simulink library "filters_lib"  (R2018b)
settings: Solver=VariableStepAuto  StartTime=0.0  StopTime=10.0  RelTol=1e-3
undefined symbols (not defined in the file or in its folder): DiscIntNeverNeededParam
libraries: quatAttitudeController_lib x1, $bdroot x1
settings Model: Creator=Ybeyer  LastModifiedBy=yannic
settings DebuggingCC: LibraryContextMissingDiagnostic=none
settings SFSimCC: SimUseLocalCustomCode=off
settings RTWCC: RTWUseLocalCustomCode=off
settings CodeAppCC: StateflowObjectComments=on

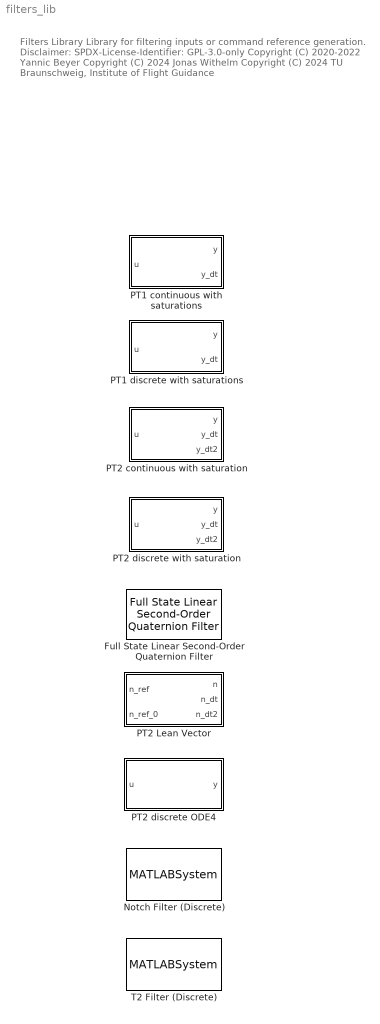
== system filters_lib ==
  note: Filters Library
      |
      | Library for filtering inputs or command reference generation.
      |
      | Disclaimer:
      | SPDX-License-Identifier: GPL-3.0-only
      |
      | Copyright (C) 2020-2022 Yannic Beyer
      | Copyright (C) 2024 Jonas Withelm
      | Copyright (C) 2024 TU Braunschweig, Institute of Flight Guidance
  Full State Linear Second-Order Quaternion Filter : quatAttitudeController_lib/Full State Linear Second-Order Quaternion Filter  omega_0=15  D=1  q_0=[1; 0; 0; 0]  omega_Kb_0=[0; 0; 0]
      settings: SourceProductName=LADAC
  Notch Filter (Discrete) : MATLABSystem  System=NotchFilter  omega_0=2*pi*80  omega_c=2*pi*40  A0_dB=40  Ts=-1  SimulateUsing=Code generation
      mask Type: NotchFilter
      mask Display:
      | disp('NotchFilter');
      | port_label('input',1,'u');
      | port_label('output',1,'y');
  PT1 continuous with saturations : Subsystem  mask{T=1, x_max=inf, x_min=-inf, x_dt_max=inf, x_dt_min=-inf, x_init=0}
      mask prompts: T "Time constant"; x_max "Maximum output"; x_min "Minimum output"; x_dt_max "Maximum output_rate"; x_dt_min "Minimum output rate"; x_init "Initial output"
  PT1 discrete with saturations : Subsystem  mask(PT1 discrete with saturation){param_src=internal, T=1, x_max=inf, x_min=-inf, x_dt_max=inf, x_dt_min=-inf, y_0_src=internal, x_init=0, is_y_dt_checked=on, is_external_reset_checked=off, mask_expr_handling_config=default}
      mask prompts: param_src "Parameter source:"; T "Time constant:"; x_max "Maximum output:"; x_min "Minimum output:"; x_dt_max "Maximum output velocity:"; x_dt_min "Minimum output velocity:"; y_0_src "Initial output source:"; x_init "Initial output:"; is_y_dt_checked "Enable velocity output"; is_external_reset_checked "Enable external reset input"
      mask init:
      | pt1BlockInit(param_src, y_0_src, is_y_dt_checked, is_external_reset_checked);
      | 
      | maskExprHandling(gcbh, mask_expr_handling_config);
      mask TypeOptions param_src: internal | external
      mask TypeOptions y_0_src: internal | external
      mask TypeOptions mask_expr_handling_config: default | passthrough (tunable)
      mask DialogControl TabGeneral Prompt: General
      mask DialogControl TabLimits Prompt: Limits
      mask DialogControl TabInitial Prompt: Initial Values
      mask DialogControl CodeGenerationSettings Prompt: Code Generation Settings
      mask DialogControl maskExprHandlingText Prompt: Mask expression handling
      mask DialogControl maskExprHandlingReadme Prompt: README
      mask DialogControl maskExprHandlingReadme Tooltip: https://github.com/iff-gsc/m-Utils/tree/main/simulink/mask_expression_handling/README.md
      mask DialogControl maskExprHandlingReadme Callback: web('https://github.com/iff-gsc/m-Utils/tree/main/simulink/mask_expression_handling/README.md','-browser')
  PT2 Lean Vector : Subsystem  mask(2nd Order Reduced Attitude Reference Model){param_src=internal, omega=1, d=1, x_max=inf, x_min=-inf, x_dt_max=inf, x_dt_min=-inf, x_dt2_max=inf, x_dt2_min=-inf, n_ref_0_src=external, x_init=[0, 0, -1], n_ref_dt_0_src=internal, x_dt_init=[0, 0, 0], is_n_dt_checked=on, is_n_dt2_checked=on, is_external_reset_checked=off, mask_expr_handling_config=default}
      mask prompts: param_src "Parameter source:"; omega "Natural frequency:"; d "Damping ratio:"; x_max "Maximum output:"; x_min "Minimum output:"; x_dt_max "Maximum output velocity:"; x_dt_min "Minimum output velocity:"; x_dt2_max "Maximum output acceleration:"; x_dt2_min "Minimum output acceleration:"; n_ref_0_src "Initial lean vector source:"; x_init "Initial lean vector:"; n_ref_dt_0_src "Initial velocity source:"; x_dt_init "Initial velocity:"; is_n_dt_checked "Enable velocity output"; is_n_dt2_checked "Enable acceleration output"; is_external_reset_checked "Enable external reset input"
      mask help: The lean vector is filtered by a second order low-pass filter. A unit vector output is assured. Moreover, the derivatives are also adjusted to match with the output unit vector.
      mask init:
      | pt2LeanVectorBlockInit(param_src, n_ref_0_src, n_ref_dt_0_src, is_n_dt_checked, is_n_dt2_checked, is_external_reset_checked);
      | 
      | maskExprHandling(gcbh, mask_expr_handling_config);
      mask TypeOptions param_src: internal | external
      mask TypeOptions n_ref_0_src: internal | external
      mask TypeOptions n_ref_dt_0_src: internal | external
      mask TypeOptions mask_expr_handling_config: default | passthrough (tunable)
      mask DialogControl TabGeneral Prompt: General
      mask DialogControl TabLimits Prompt: Limits
      mask DialogControl TabInitial Prompt: Initial Values
      mask DialogControl CodeGenerationSettings Prompt: Code Generation Settings
      mask DialogControl maskExprHandlingText Prompt: Mask expression handling
      mask DialogControl maskExprHandlingReadme Prompt: README
      mask DialogControl maskExprHandlingReadme Tooltip: https://github.com/iff-gsc/m-Utils/tree/main/simulink/mask_expression_handling/README.md
      mask DialogControl maskExprHandlingReadme Callback: web('https://github.com/iff-gsc/m-Utils/tree/main/simulink/mask_expression_handling/README.md','-browser')
  PT2 continuous with saturation : Subsystem  mask{omega=0.7, d=1, x_dt2_max=inf, x_dt2_min=-inf, x_dt_max=inf, x_dt_min=-inf, x_max=inf, x_min=-inf, x_init=0, x_dt_init=0}
      mask prompts: omega "Natural frequency"; d "Damping ratio"; x_dt2_max "Maximum acceleration"; x_dt2_min "Minimum acceleration"; x_dt_max "Maximum rate"; x_dt_min "Minimum rate"; x_max "Maximum position"; x_min "Minimum position"; x_init "Initial position"; x_dt_init "Initial rate"
  PT2 discrete ODE4 : Subsystem  mask{param_src=internal, omega=1, d=1, y_0_src=internal, x_init=0, y_dt_0_src=internal, x_dt_init=0, is_y_dt_checked=off, is_y_dt2_checked=off, is_external_reset_checked=off, mask_expr_handling_config=default}
      mask prompts: param_src "Parameter source:"; omega "Natural frequency, rad/s:"; d "Damping ratio:"; y_0_src "Initial output source:"; x_init "Initial output:"; y_dt_0_src "Initial velocity source:"; x_dt_init "Initial velocity:"; is_y_dt_checked "Enable velocity output"; is_y_dt2_checked "Enable acceleration output"; is_external_reset_checked "Enable external reset input"
      mask init:
      | pt2BlockInit(param_src, y_0_src, y_dt_0_src, is_y_dt_checked, is_y_dt2_checked, is_external_reset_checked);
      | 
      | maskExprHandling(gcbh, mask_expr_handling_config);
      mask TypeOptions param_src: internal | external
      mask TypeOptions y_0_src: internal | external
      mask TypeOptions y_dt_0_src: internal | external
      mask TypeOptions mask_expr_handling_config: default | passthrough (tunable)
      mask DialogControl DescGroupVar Prompt: Discrete second-order low-pass filter with ODE4 implementation
      mask DialogControl DescTextVar Prompt: This is a discrete second-order low-pass filter implementation with Runge-Kutta (ODE4) integration method. This method is more accurate than the standard Euler forward method (ODE1) and can be useful if the cut-off frequency is high and the sampling frequency is low.
      mask DialogControl TabGeneral Prompt: General
      mask DialogControl TabInitial Prompt: Initial Values
      mask DialogControl CodeGenerationSettings Prompt: CodeGenerationSettings
      mask DialogControl maskExprHandlingText Prompt: Mask expression handling
      mask DialogControl maskExprHandlingReadme Prompt: README
  PT2 discrete with saturation : Subsystem  mask(PT2 discrete with saturation){param_src=internal, omega=1, d=0.7, x_max=inf, x_min=-inf, x_dt_max=inf, x_dt_min=-inf, x_dt2_max=inf, x_dt2_min=-inf, y_0_src=internal, x_init=0, y_dt_0_src=internal, x_dt_init=0, is_y_dt_checked=on, is_y_dt2_checked=on, is_external_reset_checked=off, mask_expr_handling_config=default}
      mask prompts: param_src "Parameter source:"; omega "Natural frequency:"; d "Damping ratio:"; x_max "Maximum output:"; x_min "Minimum output:"; x_dt_max "Maximum output velocity:"; x_dt_min "Minimum output velocity:"; x_dt2_max "Maximum output acceleration:"; x_dt2_min "Minimum output acceleration:"; y_0_src "Initial output source:"; x_init "Initial output:"; y_dt_0_src "Initial velocity source:"; x_dt_init "Initial velocity:"; is_y_dt_checked "Enable velocity output"; is_y_dt2_checked "Enable acceleration output"; is_external_reset_checked "Enable external reset input"
      mask init:
      | pt2BlockInit(param_src, y_0_src, y_dt_0_src, is_y_dt_checked, is_y_dt2_checked, is_external_reset_checked);
      | 
      | maskExprHandling(gcbh, mask_expr_handling_config);
      mask TypeOptions param_src: internal | external
      mask TypeOptions y_0_src: internal | external
      mask TypeOptions y_dt_0_src: internal | external
      mask TypeOptions mask_expr_handling_config: default | passthrough (tunable)
      mask DialogControl TabGeneral Prompt: General
      mask DialogControl TabLimits Prompt: Limits
      mask DialogControl TabInitial Prompt: Initial Values
      mask DialogControl CodeGenerationSettings Prompt: Code Generation Settings
      mask DialogControl maskExprHandlingText Prompt: Mask expression handling
      mask DialogControl maskExprHandlingReadme Prompt: README
      mask DialogControl maskExprHandlingReadme Tooltip: https://github.com/iff-gsc/m-Utils/tree/main/simulink/mask_expression_handling/README.md
      mask DialogControl maskExprHandlingReadme Callback: web('https://github.com/iff-gsc/m-Utils/tree/main/simulink/mask_expression_handling/README.md','-browser')
  T2 Filter (Discrete) : MATLABSystem  System=T2Filter  omega_0=10  d=0.7  Ts=-1  is_vel=false  is_acc=false  SimulateUsing=Code generation
      mask Type: T2Filter
      mask Display:
      | disp('T2Filter');
      | port_label('input',1,'u');
      | port_label('output',1,'y');

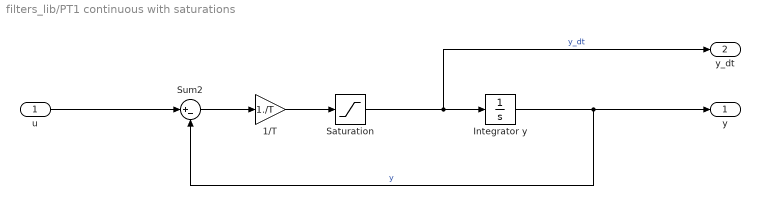
== system filters_lib/PT1 continuous with saturations ==
  u : Inport
  1/T : Gain  Gain=1./T
  Integrator y : Integrator  InitialCondition=x_init  LimitOutput=on  UpperSaturationLimit=x_max  LowerSaturationLimit=x_min
  Saturation : Saturate  UpperLimit=x_dt_max  LowerLimit=x_dt_min
  Sum2 : Sum  Inputs=|+-
  y : Outport
  y_dt : Outport  Port=2
  wires:
  Saturation/1 -> Integrator y/1, y_dt/1  "y_dt"
  Integrator y/1 -> y/1, Sum2/2  "y"
  Sum2/1 -> 1/T/1
  u/1 -> Sum2/1
  1/T/1 -> Saturation/1

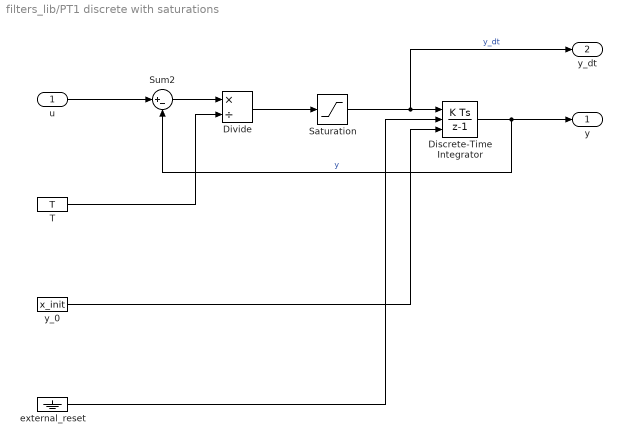
== system filters_lib/PT1 discrete with saturations ==
  u : Inport
  Discrete-Time Integrator : DiscreteIntegrator  ExternalReset=rising  InitialConditionSource=external  InitialCondition=x_init  SampleTime=-1  LimitOutput=on  UpperSaturationLimit=x_max  LowerSaturationLimit=x_min  ICPrevOutput=DiscIntNeverNeededParam  ICPrevScaledInput=DiscIntNeverNeededParam
  Divide : Product  Inputs=*/
  Saturation : Saturate  UpperLimit=x_dt_max  LowerLimit=x_dt_min
  Sum2 : Sum  Inputs=|+-
  T : Constant  Value=T
  external_reset : Ground
  y_0 : Constant  Value=x_init
  y : Outport
  y_dt : Outport  Port=2
  wires:
  Saturation/1 -> y_dt/1, Discrete-Time Integrator/1  "y_dt"
  Discrete-Time Integrator/1 -> y/1, Sum2/2  "y"
  Sum2/1 -> Divide/1
  u/1 -> Sum2/1
  Divide/1 -> Saturation/1
  T/1 -> Divide/2
  y_0/1 -> Discrete-Time Integrator/3
  external_reset/1 -> Discrete-Time Integrator/2

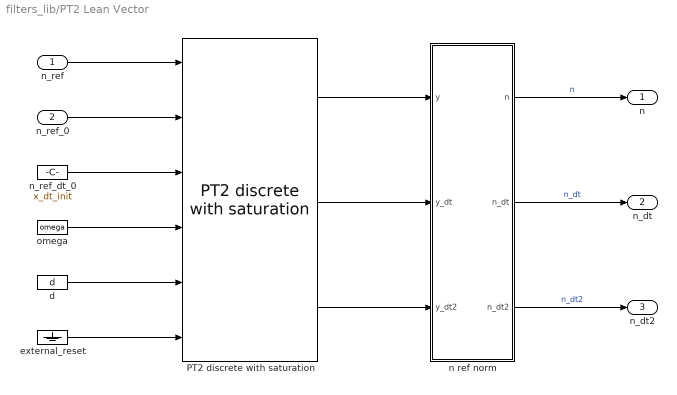
== system filters_lib/PT2 Lean Vector ==
  n_ref : Inport  PortDimensions=3
  n_ref_0 : Inport  Port=2  PortDimensions=3
  PT2 discrete with saturation : $bdroot/PT2 discrete with saturation  param_src=external  omega=omega  d=d  x_max=x_max  x_min=x_min  x_dt_max=x_dt_max  x_dt_min=x_dt_min  x_dt2_max=x_dt2_max  x_dt2_min=x_dt2_min  y_0_src=external  x_init=n_ref_0_src  y_dt_0_src=external  x_dt_init=n_ref_dt_0_src  is_y_dt_checked=on  is_y_dt2_checked=on  is_external_reset_checked=on  mask_expr_handling_config=default
  d : Constant  Value=d
  external_reset : Ground
  n ref norm : MATLAB Function  TreatAsAtomicUnit=on
  n_ref_dt_0 : Constant  Value=x_dt_init
  omega : Constant  Value=omega
  n : Outport  PortDimensions=3
  n_dt : Outport  Port=2  PortDimensions=3
  n_dt2 : Outport  Port=3  PortDimensions=3
  wires:
  n ref norm/3(n_dt2) -> n_dt2/1  "n_dt2"
  n ref norm/2(n_dt) -> n_dt/1  "n_dt"
  n ref norm/1(n) -> n/1  "n"
  PT2 discrete with saturation/1 -> n ref norm/1(y)
  PT2 discrete with saturation/2 -> n ref norm/2(y_dt)
  PT2 discrete with saturation/3 -> n ref norm/3(y_dt2)
  n_ref/1 -> PT2 discrete with saturation/1
  d/1 -> PT2 discrete with saturation/5
  omega/1 -> PT2 discrete with saturation/4
  n_ref_dt_0/1 -> PT2 discrete with saturation/3
  n_ref_0/1 -> PT2 discrete with saturation/2
  external_reset/1 -> PT2 discrete with saturation/6

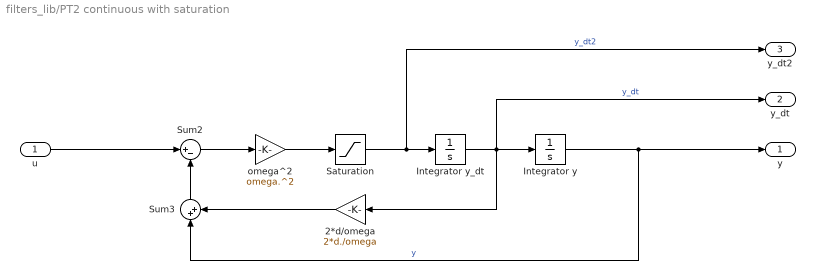
== system filters_lib/PT2 continuous with saturation ==
  u : Inport
  2*d/omega : Gain  Gain=2*d./omega
  Integrator y : Integrator  InitialCondition=x_init  LimitOutput=on  UpperSaturationLimit=x_max  LowerSaturationLimit=x_min
  Integrator y_dt : Integrator  InitialCondition=x_dt_init  LimitOutput=on  UpperSaturationLimit=x_dt_max  LowerSaturationLimit=x_dt_min
  Saturation : Saturate  UpperLimit=x_dt2_max  LowerLimit=x_dt2_min
  Sum2 : Sum  Inputs=|+-
  Sum3 : Sum  Inputs=|++
  omega^2 : Gain  Gain=omega.^2
  y : Outport
  y_dt : Outport  Port=2
  y_dt2 : Outport  Port=3
  wires:
  Integrator y_dt/1 -> y_dt/1, Integrator y/1, 2*d/omega/1  "y_dt"
  Integrator y/1 -> y/1, Sum3/1  "y"
  Sum2/1 -> omega^2/1
  2*d/omega/1 -> Sum3/2
  u/1 -> Sum2/1
  Sum3/1 -> Sum2/2
  omega^2/1 -> Saturation/1
  Saturation/1 -> y_dt2/1, Integrator y_dt/1  "y_dt2"

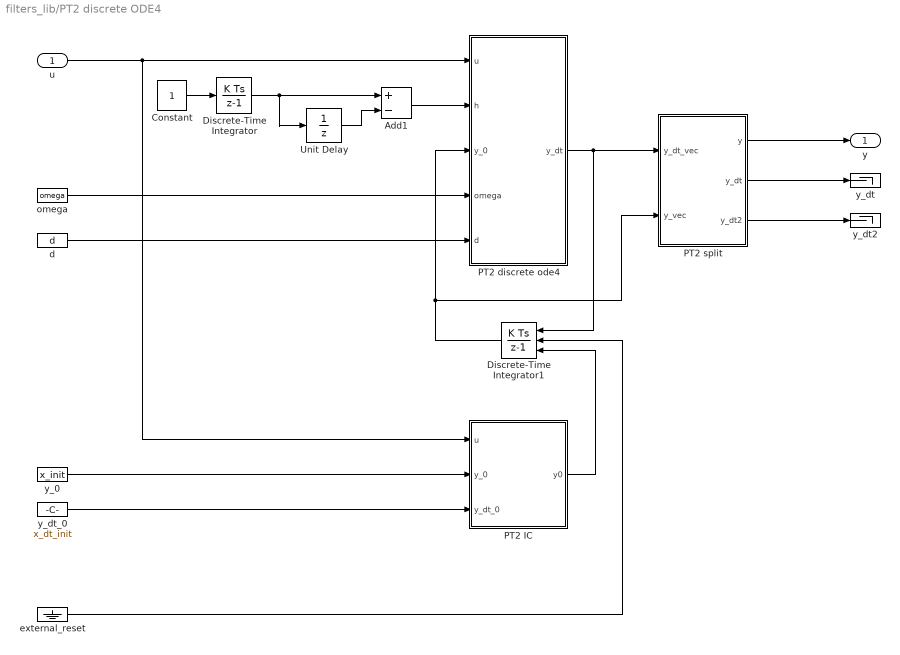
== system filters_lib/PT2 discrete ODE4 ==
  u : Inport
  Add1 : Sum  Inputs=+-
  Constant : Constant
  Discrete-Time Integrator : DiscreteIntegrator  SampleTime=-1  ICPrevOutput=DiscIntNeverNeededParam  ICPrevScaledInput=DiscIntNeverNeededParam
  Discrete-Time Integrator1 : DiscreteIntegrator  ExternalReset=rising  InitialConditionSource=external  SampleTime=-1  ICPrevOutput=DiscIntNeverNeededParam  ICPrevScaledInput=DiscIntNeverNeededParam
  PT2 IC : MATLAB Function  TreatAsAtomicUnit=on
  PT2 discrete ode4 : MATLAB Function  TreatAsAtomicUnit=on
  PT2 split : MATLAB Function  TreatAsAtomicUnit=on
  Unit Delay : UnitDelay  SampleTime=-1
  d : Constant  Value=d
  external_reset : Ground
  omega : Constant  Value=omega
  y_0 : Constant  Value=x_init
  y_dt : Terminator
  y_dt2 : Terminator
  y_dt_0 : Constant  Value=x_dt_init
  y : Outport
  wires:
  u/1 -> PT2 IC/1(u), PT2 discrete ode4/1(u)
  Constant/1 -> Discrete-Time Integrator/1
  Add1/1 -> PT2 discrete ode4/2(h)
  Discrete-Time Integrator/1 -> Add1/1, Unit Delay/1
  Unit Delay/1 -> Add1/2
  omega/1 -> PT2 discrete ode4/4(omega)
  d/1 -> PT2 discrete ode4/5(d)
  PT2 discrete ode4/1(y_dt) -> Discrete-Time Integrator1/1, PT2 split/1(y_dt_vec)
  Discrete-Time Integrator1/1 -> PT2 split/2(y_vec), PT2 discrete ode4/3(y_0)
  PT2 split/1(y) -> y/1
  PT2 split/2(y_dt) -> y_dt/1
  PT2 split/3(y_dt2) -> y_dt2/1
  y_0/1 -> PT2 IC/2(y_0)
  y_dt_0/1 -> PT2 IC/3(y_dt_0)
  external_reset/1 -> Discrete-Time Integrator1/2
  PT2 IC/1(y0) -> Discrete-Time Integrator1/3

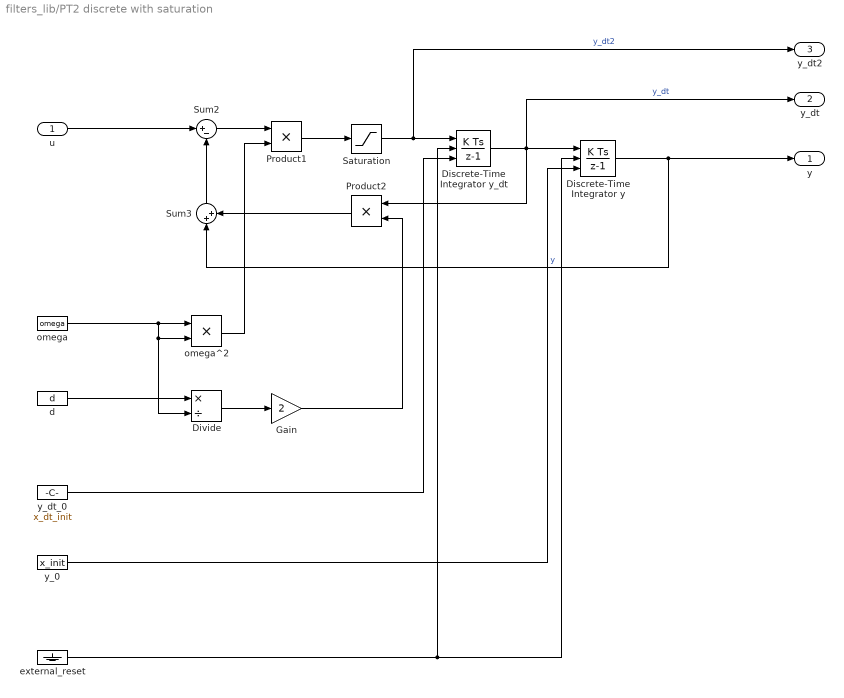
== system filters_lib/PT2 discrete with saturation ==
  u : Inport
  Discrete-Time Integrator y : DiscreteIntegrator  ExternalReset=rising  InitialConditionSource=external  InitialCondition=x_init  SampleTime=-1  LimitOutput=on  UpperSaturationLimit=x_max  LowerSaturationLimit=x_min  ICPrevOutput=DiscIntNeverNeededParam  ICPrevScaledInput=DiscIntNeverNeededParam
  Discrete-Time Integrator y_dt : DiscreteIntegrator  ExternalReset=rising  InitialConditionSource=external  InitialCondition=x_dt_init  SampleTime=-1  LimitOutput=on  UpperSaturationLimit=x_dt_max  LowerSaturationLimit=x_dt_min  ICPrevOutput=DiscIntNeverNeededParam  ICPrevScaledInput=DiscIntNeverNeededParam
  Divide : Product  Inputs=*/
  Gain : Gain  Gain=2
  Product1 : Product
  Product2 : Product
  Saturation : Saturate  UpperLimit=x_dt2_max  LowerLimit=x_dt2_min
  Sum2 : Sum  Inputs=|+-
  Sum3 : Sum  Inputs=|++
  d : Constant  Value=d
  external_reset : Ground
  omega : Constant  Value=omega
  omega^2 : Product
  y_0 : Constant  Value=x_init
  y_dt_0 : Constant  Value=x_dt_init
  y : Outport
  y_dt : Outport  Port=2
  y_dt2 : Outport  Port=3
  wires:
  Discrete-Time Integrator y_dt/1 -> Product2/1, Discrete-Time Integrator y/1, y_dt/1  "y_dt"
  Discrete-Time Integrator y/1 -> y/1, Sum3/1  "y"
  Sum2/1 -> Product1/1
  Product2/1 -> Sum3/2
  u/1 -> Sum2/1
  Sum3/1 -> Sum2/2
  Product1/1 -> Saturation/1
  Saturation/1 -> Discrete-Time Integrator y_dt/1, y_dt2/1  "y_dt2"
  y_0/1 -> Discrete-Time Integrator y/3
  y_dt_0/1 -> Discrete-Time Integrator y_dt/3
  omega/1 -> Divide/2, omega^2/2, omega^2/1
  omega^2/1 -> Product1/2
  Divide/1 -> Gain/1
  d/1 -> Divide/1
  Gain/1 -> Product2/2
  external_reset/1 -> Discrete-Time Integrator y/2, Discrete-Time Integrator y_dt/2

== matlab function filters_lib/PT2 discrete ODE4/PT2 IC ==
  data: u input; y0 output; y_0 input; y_dt_0 input
function y0 = fcn(u, y_0, y_dt_0)
y0 = zeros([2,size(u)],class(u));
y0(1,:) = y_dt_0;
y0(2,:) = y_0;
end

== matlab function filters_lib/PT2 Lean Vector/n ref norm ==
  data: y input; y_dt input; n output; n_dt output; n_dt2 output; y_dt2 input
function [n, n_dt, n_dt2] = fcn(y, y_dt, y_dt2)

norm_n  = norm(y,2);
n       = divideFinite( y, norm_n );

n_dt    = leanVectorNormDeriv(y,y_dt);
n_dt2   = leanVectorNormDeriv2(y,y_dt,y_dt2);

end

== matlab function filters_lib/PT2 discrete ODE4/PT2 discrete ode4 ==
  data: y_dt output; u input; h input; y_0 input; omega input; d input
function y_dt  = fcn(u, h, y_0, omega, d)

y_dt = zeros([2,size(u)],class(u));

% y = [y_dt_0;y_0];

k1 = f(y_0,u,omega,d);
k2 = f(y_0+0.5*h*k1,u,omega,d);
k3 = f(y_0+0.5*h*k2,u,omega,d);
k4 = f(y_0+h*k3,u,omega,d);

y_dt(:) = 1/6*(k1+2*k2+2*k3+k4);
% y_dt2(:) = 1/6*(k1(1,:)+2*k2(1,:)+2*k3(1,:)+k4(1,:));

function y_vec_dt = f(y_0,u,omega,d)
    len_u = length(u);
    y_vec_dt = zeros(2,len_u,superiorfloat(u));
%     y_vec_dt = zeros(1,len_u,class(u));
    for i = 1:len_u
        y_vec_dt(:,i) = [ -2*d*omega, -omega^2; 1, 0 ] * y_0(:,i) + [omega^2;0] * u(i);
%         y_vec_dt(i) = [ -2*d*omega, -omega^2 ] * y_0(:,i) + omega^2 * u(i);
    end
end

end

== matlab function filters_lib/PT2 discrete ODE4/PT2 split ==
  data: y_dt_vec input; y_vec input; y output; y_dt output; y_dt2 output
function [y,y_dt,y_dt2] = fcn(y_dt_vec, y_vec)
y = y_vec(2,:)';
y_dt = y_dt_vec(2,:)';
y_dt2 = y_dt_vec(1,:)';
end
